simulink model "Prj2CDig_discreto_PRJ2"  (R2026b)
settings: Solver=FixedStepDiscrete  StopTime=3600  FixedStep=5.7149999999999999  RelTol=1e-6  EnableMultiTasking=on
model workspace (MAT data in the model file):
  C_Tustin = 2.8575
  C_seno_1 = 1.30135744433
  C_seno_2 = 5.41983902077
  G_termico_PWM16 = 455.852369272
  K_AW = 0.0178971363858
  K_obs_1 = 2.42292827366
  K_obs_2 = 37.30035107
  K_obs_q = 0.454670555849
  Ki = 55.874860561
  Nb = 1615.01542842
  Ta0 = 26.5945354915
  u0 = 9688.13559322
  y0 = 50.50283
settings Model: Creator=Adolfo  LastModifiedBy=Santana
settings SolverCC: ZeroCrossControl=DisableAll
settings DataIOCC: LimitDataPoints=on  MaxDataPoints=25000  SaveFormat=Array  SignalLoggingSaveFormat=ModelDataLogs
settings OptimizationCC: BlockReduction=off  BooleanDataType=off  LifeSpan=inf  MemsetInitFltsAndDblsToZero=off  ReuseModelBlockBuffer=off
settings DebuggingCC: ArithmeticOperatorsInVariantConditions=warning  FcnCallInpInsideContextMsg=warning  MergeDetectMultiDrivingBlocksExec=none  MultiTaskCondExecSysMsg=none  MultiTaskDSMMsg=warning  SFExecutionAtInitializationDiag=none  SFNoUnconditionalDefaultTransitionDiag=warning  SFUnexpectedBacktrackingDiag=warning  SaveWithParameterizedLinksMsg=none  SignalResolutionControl=TryResolveAllWithWarning  StateNameClashWarn=warning
settings HardwareCC: ProdEndianess=Unspecified  ProdHWDeviceType=32-bit Generic  ProdIntDivRoundTo=Undefined  ProdLargestAtomicFloat=None  TargetUnknown=on
settings ModelReferenceCC: PropagateSignalLabelsOutOfModel=off
settings SFSimCC: CustomCodeUndefinedFunction=UseInterfaceOnly  SimUseLocalCustomCode=off
settings RTWCC: RTWUseLocalCustomCode=off
settings CodeAppCC: StateflowObjectComments=on
settings GRTTargetCC: CombineOutputUpdateFcns=off  GRTInterface=on  TargetFcnLib=ansi_tfl_tmw.mat  TargetLangStandard=C89/C90 (ANSI)
settings ConfigComp: CovSaveCumulativeToWorkspaceVar=on  CovSaveSingleToWorkspaceVar=on

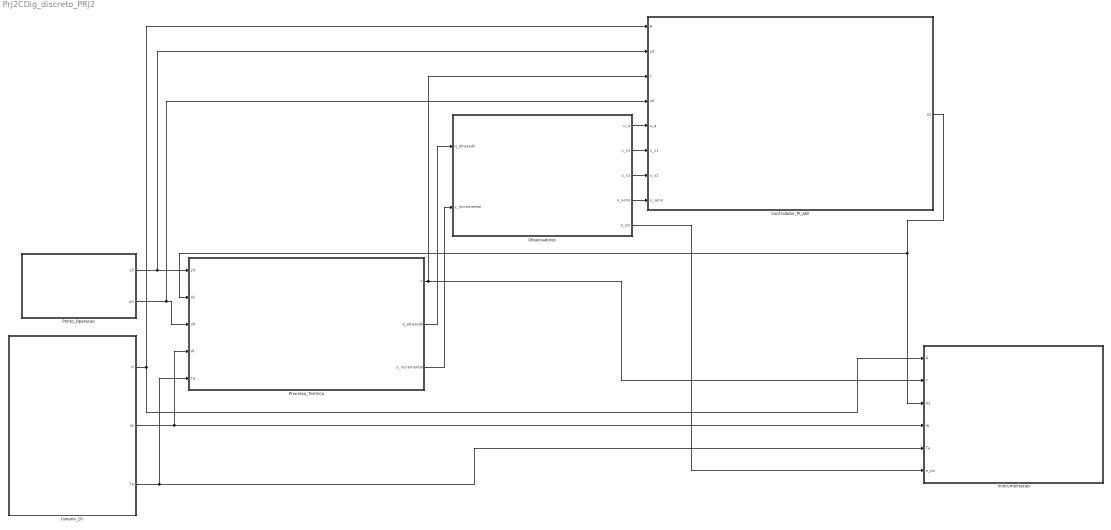
== system Prj2CDig_discreto_PRJ2 ==
  Cenario_1h : Subsystem
  Controlador_PI_AW : Subsystem
  Instrumentacao : Subsystem
  Observadores : Subsystem
  Ponto_Operacao : Subsystem
  Processo_Termico : Subsystem
  wires:
  Processo_Termico/3(y_incremental) -> Observadores/2(y_incremental)
  Processo_Termico/2(q_atrasado) -> Observadores/1(q_atrasado)
  Processo_Termico/1(Y) -> Instrumentacao/2(Y), Controlador_PI_AW/3(Y)
  Ponto_Operacao/2(u0) -> Controlador_PI_AW/4(u0), Processo_Termico/3(u0)
  Ponto_Operacao/1(y0) -> Processo_Termico/1(y0), Controlador_PI_AW/2(y0)
  Cenario_1h/2(W) -> Instrumentacao/4(W), Processo_Termico/4(W)
  Cenario_1h/1(R) -> Instrumentacao/1(R), Controlador_PI_AW/1(R)
  Observadores/1(u_q) -> Controlador_PI_AW/5(u_q)
  Cenario_1h/3(Ta) -> Instrumentacao/5(Ta), Processo_Termico/5(Ta)
  Observadores/2(u_x1) -> Controlador_PI_AW/6(u_x1)
  Observadores/3(u_x2) -> Controlador_PI_AW/7(u_x2)
  Observadores/4(u_seno) -> Controlador_PI_AW/8(u_seno)
  Observadores/5(e_sin) -> Instrumentacao/6(e_sin)
  Controlador_PI_AW/1(Us) -> Instrumentacao/3(Us), Processo_Termico/2(Us)

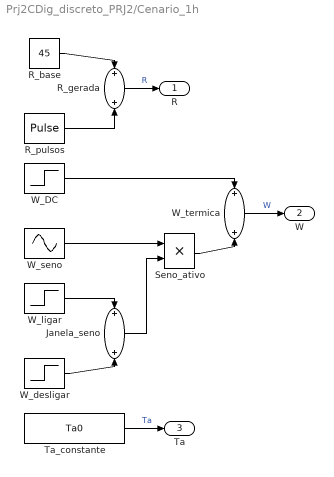
== system Prj2CDig_discreto_PRJ2/Cenario_1h ==
  Janela_seno : Sum
  R_base : Constant  Value=45
  R_gerada : Sum
  R_pulsos : DiscretePulseGenerator  Amplitude=10  Period=140  PulseWidth=70  PhaseDelay=70  SampleTime=5.7149999999999999
  Seno_ativo : Product
  Ta_constante : Constant  Value=Ta0
  W_DC : Step  Time=1000  FinalValue=-20  SampleTime=5.7149999999999999
  W_desligar : Step  Time=3000  FinalValue=-1  SampleTime=5.7149999999999999
  W_ligar : Step  Time=1800  SampleTime=5.7149999999999999
  W_seno : Sin  Amplitude=20  Frequency=0.098174770424681035  Phase=-176.71458676442586  SampleTime=5.7149999999999999
  W_termica : Sum
  R : Outport
  W : Outport  Port=2
  Ta : Outport  Port=3
  wires:
  R_pulsos/1 -> R_gerada/2
  R_gerada/1 -> R/1  "R"
  R_base/1 -> R_gerada/1
  W_desligar/1 -> Janela_seno/2
  W_termica/1 -> W/1  "W"
  W_ligar/1 -> Janela_seno/1
  W_seno/1 -> Seno_ativo/1
  Ta_constante/1 -> Ta/1  "Ta"
  Janela_seno/1 -> Seno_ativo/2
  W_DC/1 -> W_termica/1
  Seno_ativo/1 -> W_termica/2

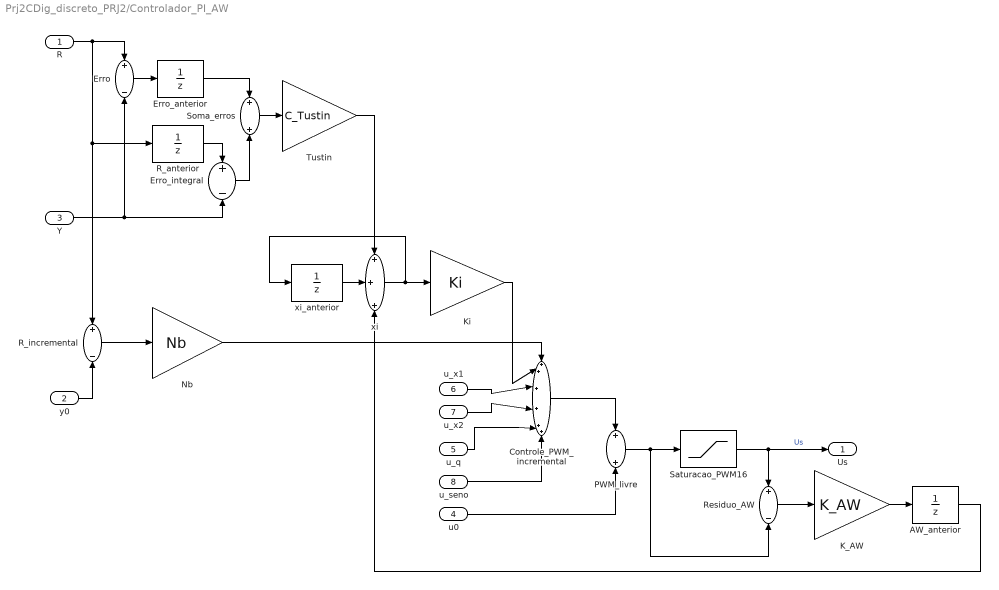
== system Prj2CDig_discreto_PRJ2/Controlador_PI_AW ==
  R : Inport
  y0 : Inport  Port=2
  Y : Inport  Port=3
  u0 : Inport  Port=4
  u_q : Inport  Port=5
  u_x1 : Inport  Port=6
  u_x2 : Inport  Port=7
  u_seno : Inport  Port=8
  AW_anterior : UnitDelay  SampleTime=5.7149999999999999
  Controle_PWM_incremental : Sum  Inputs=++++++
  Erro : Sum  Inputs=+-
  Erro_anterior : UnitDelay  SampleTime=5.7149999999999999
  Erro_integral : Sum  Inputs=+-
  K_AW : Gain  Gain=K_AW
  Ki : Gain  Gain=Ki
  Nb : Gain  Gain=Nb
  PWM_livre : Sum
  R_anterior : UnitDelay  InitialCondition=50  SampleTime=5.7149999999999999
  R_incremental : Sum  Inputs=+-
  Residuo_AW : Sum  Inputs=+-
  Saturacao_PWM16 : Saturate  UpperLimit=65535  LowerLimit=0
  Soma_erros : Sum
  Tustin : Gain  Gain=C_Tustin
  xi : Sum  Inputs=+++
  xi_anterior : UnitDelay  InitialCondition=-7.5988805980816405  SampleTime=5.7149999999999999
  Us : Outport
  wires:
  R/1 -> Erro/1, R_anterior/1, R_incremental/1
  Erro/1 -> Erro_anterior/1
  Y/1 -> Erro_integral/2, Erro/2
  u_seno/1 -> Controle_PWM_incremental/6
  y0/1 -> R_incremental/2
  R_anterior/1 -> Erro_integral/1
  Residuo_AW/1 -> K_AW/1
  R_incremental/1 -> Nb/1
  Soma_erros/1 -> Tustin/1
  Nb/1 -> Controle_PWM_incremental/1
  Tustin/1 -> xi/1
  xi_anterior/1 -> xi/2
  xi/1 -> Ki/1, xi_anterior/1
  u_x2/1 -> Controle_PWM_incremental/4
  u_q/1 -> Controle_PWM_incremental/5
  Ki/1 -> Controle_PWM_incremental/2
  u_x1/1 -> Controle_PWM_incremental/3
  u0/1 -> PWM_livre/2
  AW_anterior/1 -> xi/3
  Controle_PWM_incremental/1 -> PWM_livre/1
  PWM_livre/1 -> Saturacao_PWM16/1, Residuo_AW/2
  Saturacao_PWM16/1 -> Us/1, Residuo_AW/1  "Us"
  K_AW/1 -> AW_anterior/1
  Erro_anterior/1 -> Soma_erros/1
  Erro_integral/1 -> Soma_erros/2

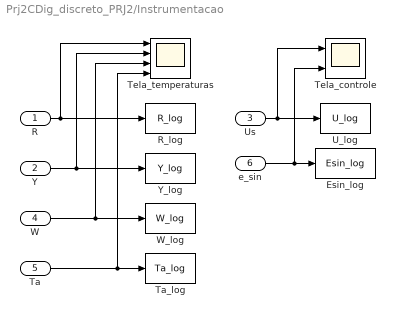
== system Prj2CDig_discreto_PRJ2/Instrumentacao ==
  R : Inport
  Y : Inport  Port=2
  Us : Inport  Port=3
  W : Inport  Port=4
  Ta : Inport  Port=5
  e_sin : Inport  Port=6
  Esin_log : ToWorkspace  VariableName=Esin_log  SaveFormat=Timeseries  SampleTime=-1
  R_log : ToWorkspace  VariableName=R_log  SaveFormat=Timeseries  SampleTime=-1
  Ta_log : ToWorkspace  VariableName=Ta_log  SaveFormat=Timeseries  SampleTime=-1
  Tela_controle : Scope  NumInputPorts=2
      settings: Title=Controle e compensacao - simulacao discreta (1 h)  ActiveDisplayYMinimum=-11304.641937639226  ActiveDisplayYMaximum=46291.484135415289  YLabel=PWM16
  Tela_temperaturas : Scope  NumInputPorts=4
      settings: Title=Temperaturas e perturbacao - simulacao discreta (1 h)  ActiveDisplayYMinimum=-52.429435518981052  ActiveDisplayYMaximum=71.927589349427066  YLabel=Temperatura / W (graus C)
  U_log : ToWorkspace  VariableName=U_log  SaveFormat=Timeseries  SampleTime=-1
  W_log : ToWorkspace  VariableName=W_log  SaveFormat=Timeseries  SampleTime=-1
  Y_log : ToWorkspace  VariableName=Y_log  SaveFormat=Timeseries  SampleTime=-1
  wires:
  W/1 -> W_log/1, Tela_temperaturas/3
  Y/1 -> Y_log/1, Tela_temperaturas/2
  Us/1 -> Tela_controle/1, U_log/1
  e_sin/1 -> Tela_controle/2, Esin_log/1
  R/1 -> R_log/1, Tela_temperaturas/1
  Ta/1 -> Ta_log/1, Tela_temperaturas/4

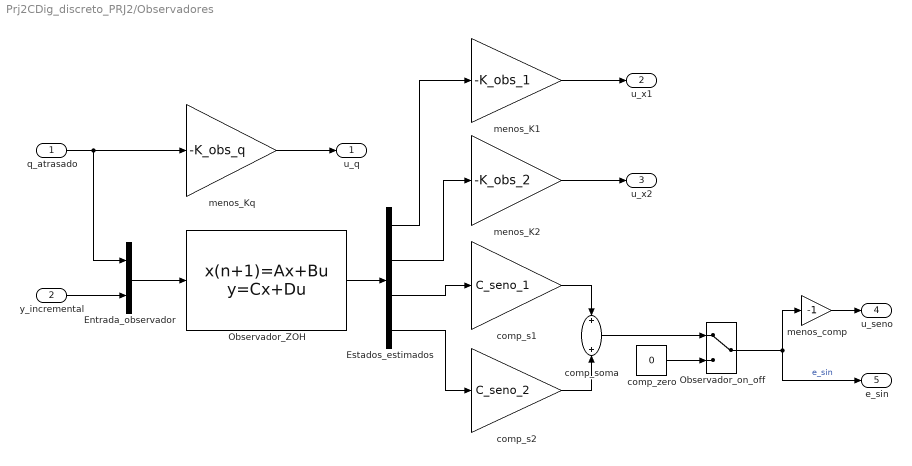
== system Prj2CDig_discreto_PRJ2/Observadores ==
  q_atrasado : Inport
  y_incremental : Inport  Port=2
  Entrada_observador : Mux  Inputs=2
  Estados_estimados : Demux
  Observador_ZOH : DiscreteStateSpace  A=[0.87148850627135255 -2.3349292179027987 0.012391015895003424 0;-0.021460368525439675 0.36223061019376079 0.011491559879183539 0;0.54700065839072487 12.12681339185988 0.84668688848431295 5.4198390207695537;0.098868116531183062 2.1918715840409377 -0.052237956106038111 0.84668688848431295]  B=[0.012391015895003424 101.15520303030875;0.011491559879183539 20.611544085060167;0 -525.365078032665;0 -94.957574473786678]  C=[1 0 0 0;0 1 0 0;0 0 1 0;0 0 0 1]  D=[0 0;0 0;0 0;0 0]  InitialCondition=[-122.47342486472;-16.259529340423821;0;0]  SampleTime=5.7149999999999999
  Observador_on_off : ManualSwitch
  comp_s1 : Gain  Gain=C_seno_1
  comp_s2 : Gain  Gain=C_seno_2
  comp_soma : Sum
  comp_zero : Constant  Value=0
  menos_K1 : Gain  Gain=-K_obs_1
  menos_K2 : Gain  Gain=-K_obs_2
  menos_Kq : Gain  Gain=-K_obs_q
  menos_comp : Gain  Gain=-1
  u_q : Outport
  u_x1 : Outport  Port=2
  u_x2 : Outport  Port=3
  u_seno : Outport  Port=4
  e_sin : Outport  Port=5
  wires:
  q_atrasado/1 -> menos_Kq/1, Entrada_observador/1
  Entrada_observador/1 -> Observador_ZOH/1
  y_incremental/1 -> Entrada_observador/2
  Estados_estimados/3 -> comp_s1/1
  Estados_estimados/2 -> menos_K2/1
  Estados_estimados/1 -> menos_K1/1
  menos_Kq/1 -> u_q/1
  Observador_on_off/1 -> menos_comp/1, e_sin/1  "e_sin"
  Observador_ZOH/1 -> Estados_estimados/1
  Estados_estimados/4 -> comp_s2/1
  comp_s1/1 -> comp_soma/1
  menos_K1/1 -> u_x1/1
  menos_K2/1 -> u_x2/1
  comp_soma/1 -> Observador_on_off/1
  comp_s2/1 -> comp_soma/2
  comp_zero/1 -> Observador_on_off/2
  menos_comp/1 -> u_seno/1

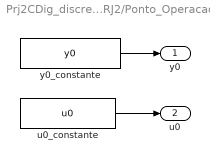
== system Prj2CDig_discreto_PRJ2/Ponto_Operacao ==
  u0_constante : Constant  Value=u0
  y0_constante : Constant  Value=y0
  y0 : Outport
  u0 : Outport  Port=2
  wires:
  y0_constante/1 -> y0/1
  u0_constante/1 -> u0/1

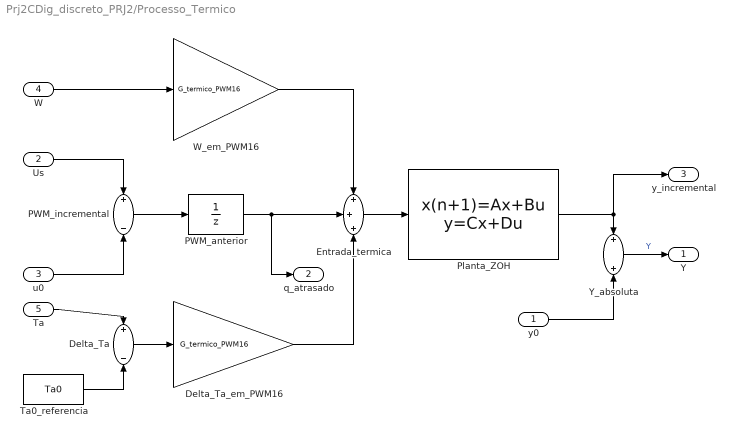
== system Prj2CDig_discreto_PRJ2/Processo_Termico ==
  y0 : Inport
  Us : Inport  Port=2
  u0 : Inport  Port=3
  W : Inport  Port=4
  Ta : Inport  Port=5
  Delta_Ta : Sum  Inputs=+-
  Delta_Ta_em_PWM16 : Gain  Gain=G_termico_PWM16
  Entrada_termica : Sum  Inputs=+++
  PWM_anterior : UnitDelay  InitialCondition=-229.21624684123856  SampleTime=5.7149999999999999
  PWM_incremental : Sum  Inputs=+-
  Planta_ZOH : DiscreteStateSpace  A=[0.97680948204771745 0;0 0.83799947890809312]  B=[0.012391015895003424;0.011491559879183539]  C=[0.0010411819918428509 0.023082640812882287]  D=0  InitialCondition=[-122.47342486472;-16.259529340423821]  SampleTime=5.7149999999999999
  Ta0_referencia : Constant  Value=Ta0
  W_em_PWM16 : Gain  Gain=G_termico_PWM16
  Y_absoluta : Sum
  Y : Outport
  q_atrasado : Outport  Port=2
  y_incremental : Outport  Port=3
  wires:
  u0/1 -> PWM_incremental/2
  Us/1 -> PWM_incremental/1
  W/1 -> W_em_PWM16/1
  PWM_incremental/1 -> PWM_anterior/1
  PWM_anterior/1 -> q_atrasado/1, Entrada_termica/2
  Entrada_termica/1 -> Planta_ZOH/1
  Planta_ZOH/1 -> y_incremental/1, Y_absoluta/1
  y0/1 -> Y_absoluta/2
  Y_absoluta/1 -> Y/1  "Y"
  Ta/1 -> Delta_Ta/1
  Ta0_referencia/1 -> Delta_Ta/2
  Delta_Ta/1 -> Delta_Ta_em_PWM16/1
  Delta_Ta_em_PWM16/1 -> Entrada_termica/3
  W_em_PWM16/1 -> Entrada_termica/1
